simulink subsystem "fft2d"  (R2024b)
settings: Solver=VariableStepAuto  StartTime=0.0  StopTime=10.0  RelTol=1e-3
undefined symbols (not defined in the file): B, L, LOG2B, LOG2L, NFR, PH_W, RAM_AW, W
libraries: hdlsllib x25, dsphdlxfrm2 x1
settings Model: Creator=User  LastModifiedBy=aaala

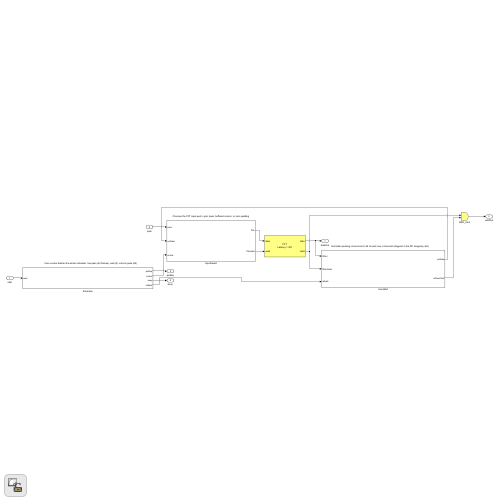
[thumbnail: Simulink's stored preview of the top-level diagram]
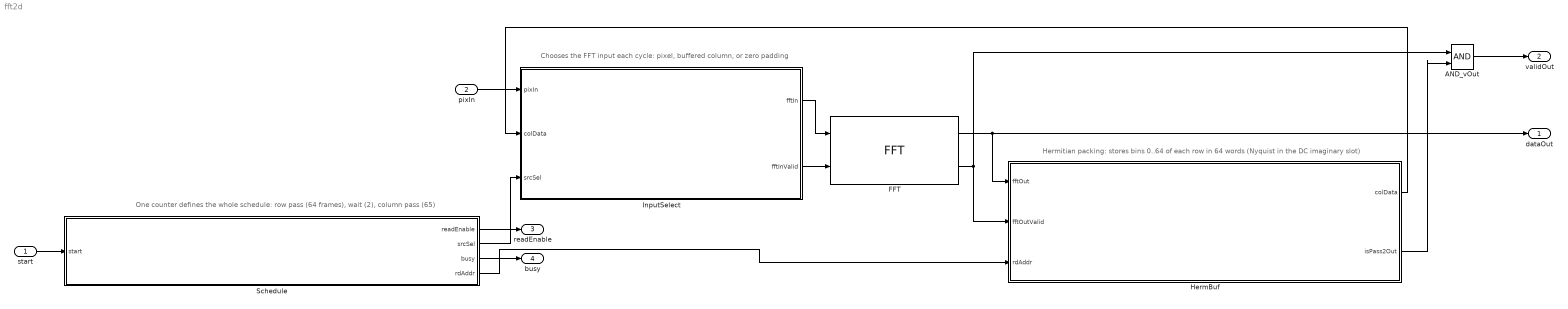
== system fft2d ==
  note: Hermitian packing: stores bins 0..64 of each row in 64 words (Nyquist in the DC imaginary slot)
  note: Chooses the FFT input each cycle: pixel, buffered column, or zero padding
  note: One counter defines the whole schedule: row pass (64 frames), wait (2), column pass (65)
  start : Inport
  pixIn : Inport  Port=2  OutDataTypeStr=uint8
  AND_vOut : Logic  IconShape=distinctive  AllPortsSameDT=off  OutDataTypeStr=boolean
  FFT : dsphdlxfrm2/FFT  Architecture=Streaming Radix 2^2  FFTLengthSource=Property  FFTLength=128  FFTLengthMax=1024  ComplexMultiplication=Use 4 multipliers and 2 adders  BitReversedOutput=off  BitReversedInput=off  Normalize=off  SimulateUsing=Code generation  RoundingMethod=Floor  ResetInputPort=off  StartOutputPort=off  EndOutputPort=off
  HermBuf : Subsystem
  InputSelect : Subsystem
  Schedule : Subsystem
  dataOut : Outport
  validOut : Outport  Port=2
  readEnable : Outport  Port=3
  busy : Outport  Port=4
  wires:
  start/1 -> Schedule/1(start)
  pixIn/1 -> InputSelect/1(pixIn)
  Schedule/3(busy) -> busy/1
  Schedule/1(readEnable) -> readEnable/1
  Schedule/2(srcSel) -> InputSelect/3(srcSel)
  InputSelect/1(fftIn) -> FFT/1
  Schedule/4(rdAddr) -> HermBuf/3(rdAddr)
  InputSelect/2(fftInValid) -> FFT/2
  FFT/1 -> HermBuf/1(fftOut), dataOut/1
  FFT/2 -> HermBuf/2(fftOutValid), AND_vOut/1
  HermBuf/1(colData) -> InputSelect/2(colData)
  HermBuf/2(isPass2Out) -> AND_vOut/2
  AND_vOut/1 -> validOut/1

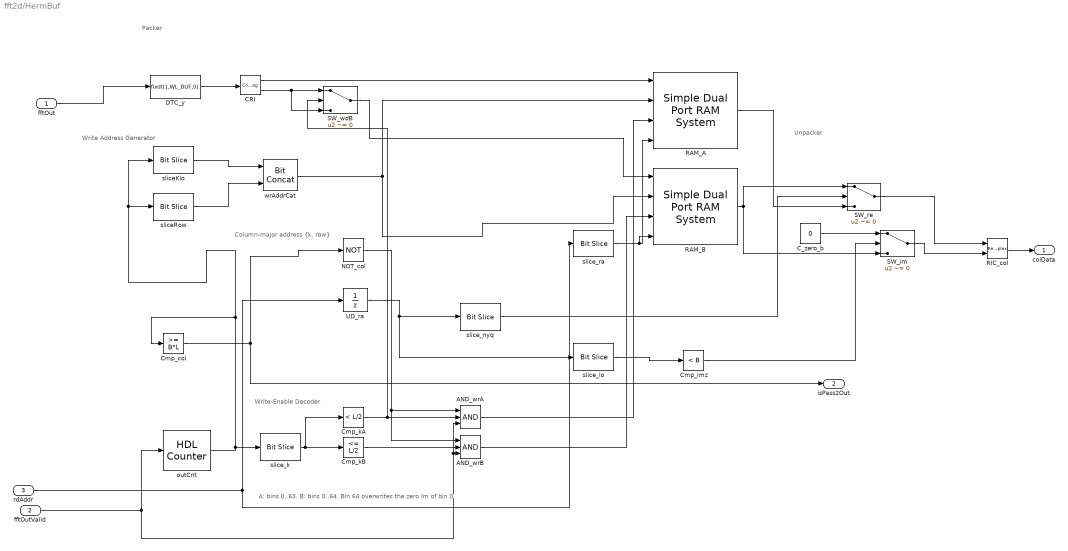
== system fft2d/HermBuf ==
  note: Write-Enable Decoder
  note: A: bins 0..63. B: bins 0..64. Bin 64 overwrites the zero Im of bin 0
  note: Write Address Generator
  note: Column-major address {k, row}
  note: Packer
  note: Unpacker
  fftOut : Inport
  fftOutValid : Inport  Port=2
  rdAddr : Inport  Port=3
  AND_wrA : Logic  Inputs=3  IconShape=distinctive  AllPortsSameDT=off  OutDataTypeStr=boolean
  AND_wrB : Logic  Inputs=3  IconShape=distinctive  AllPortsSameDT=off  OutDataTypeStr=boolean
  CRI : ComplexToRealImag
  C_zero_b : Constant  Value=0  OutDataTypeStr=fixdt(1,WL_BUF,0)
  Cmp_col : hdlsllib/Logic and Bit Operations/Compare To Constant  relop=>=  const=B*L  OutDataTypeStr=boolean
  Cmp_imz : hdlsllib/Logic and Bit Operations/Compare To Constant  relop=<  const=B  OutDataTypeStr=boolean
  Cmp_kA : hdlsllib/Logic and Bit Operations/Compare To Constant  relop=<  const=L/2  OutDataTypeStr=boolean
  Cmp_kB : hdlsllib/Logic and Bit Operations/Compare To Constant  relop=<=  const=L/2  OutDataTypeStr=boolean
  DTC_y : DataTypeConversion  OutDataTypeStr=fixdt(1,WL_BUF,0)  SaturateOnIntegerOverflow=off  RndMeth=Floor
  NOT_col : Logic  Operator=NOT  IconShape=distinctive  AllPortsSameDT=off  OutDataTypeStr=boolean
  RAM_A : hdlsllib/HDL RAMs/Simple Dual Port RAM System  RAMType=Simple dual port  AsyncRead=off  WriteOutputValue=New data  RAMInitialValue=0  allowBusInputs=off  WritesHaveOutput=on  NumReads=0  NumWrites=1  SimulateUsing=Code generation  ModelRAMDelay=on
  RAM_B : hdlsllib/HDL RAMs/Simple Dual Port RAM System  RAMType=Simple dual port  AsyncRead=off  WriteOutputValue=New data  RAMInitialValue=0  allowBusInputs=off  WritesHaveOutput=on  NumReads=0  NumWrites=1  SimulateUsing=Code generation  ModelRAMDelay=on
  RIC_col : RealImagToComplex
  SW_im : Switch  Criteria=u2 ~= 0  SaturateOnIntegerOverflow=off  InputSameDT=off
  SW_re : Switch  Criteria=u2 ~= 0  SaturateOnIntegerOverflow=off  InputSameDT=off
  SW_wdB : Switch  Criteria=u2 ~= 0  SaturateOnIntegerOverflow=off  InputSameDT=off
  UD_ra : UnitDelay  SampleTime=-1  HasFrameUpgradeWarning=on
  outCnt : hdlsllib/Sources/HDL Counter  CountType=Count limited  CountInit=0  CountStep=1  CountMax=OC_MAX  CountFromType=Initial value  CountFrom=0  CountResetPort=off  CountLoadPort=off  CountEnbPort=on  CountDirPort=off  CountHitOutputPort=off  CountDataType=Unsigned  CountWordLen=OC_W  CountFracLen=0  CountSampTime=1
  sliceKlo : hdlsllib/Logic and Bit Operations/Bit Slice  lidx=LOG2L-2  ridx=0
  sliceRow : hdlsllib/Logic and Bit Operations/Bit Slice  lidx=LOG2L+LOG2B-1  ridx=LOG2L
  slice_k : hdlsllib/Logic and Bit Operations/Bit Slice  lidx=LOG2L-1  ridx=0
  slice_lo : hdlsllib/Logic and Bit Operations/Bit Slice  lidx=RAM_AW-1  ridx=0
  slice_nyq : hdlsllib/Logic and Bit Operations/Bit Slice  lidx=RAM_AW  ridx=RAM_AW
  slice_ra : hdlsllib/Logic and Bit Operations/Bit Slice  lidx=RAM_AW-1  ridx=0
  wrAddrCat : hdlsllib/Logic and Bit Operations/Bit Concat  numInputs=2
  colData : Outport
  isPass2Out : Outport  Port=2
  wires:
  SW_im/1 -> RIC_col/2
  SW_re/1 -> RIC_col/1
  Cmp_imz/1 -> SW_im/2
  C_zero_b/1 -> SW_im/1
  RAM_B/1 -> SW_re/1, SW_im/3
  RAM_A/1 -> SW_re/3
  slice_nyq/1 -> SW_re/2
  AND_wrB/1 -> RAM_B/3
  slice_ra/1 -> RAM_B/4, RAM_A/4
  AND_wrA/1 -> RAM_A/3
  RIC_col/1 -> colData/1
  Cmp_kB/1 -> AND_wrB/2
  Cmp_kA/1 -> AND_wrA/2, SW_wdB/2
  wrAddrCat/1 -> RAM_B/2, RAM_A/2
  NOT_col/1 -> AND_wrB/1, AND_wrA/1
  CRI/2 -> SW_wdB/1, SW_wdB/3
  slice_lo/1 -> Cmp_imz/1
  CRI/1 -> RAM_A/1
  UD_ra/1 -> slice_nyq/1, slice_lo/1
  Cmp_col/1 -> isPass2Out/1, NOT_col/1
  slice_k/1 -> Cmp_kA/1, Cmp_kB/1
  DTC_y/1 -> CRI/1
  sliceRow/1 -> wrAddrCat/2
  SW_wdB/1 -> RAM_B/1
  outCnt/1 -> slice_k/1, Cmp_col/1, sliceRow/1, sliceKlo/1
  rdAddr/1 -> UD_ra/1, slice_ra/1
  fftOut/1 -> DTC_y/1
  fftOutValid/1 -> outCnt/1, AND_wrB/3, AND_wrA/3
  sliceKlo/1 -> wrAddrCat/1

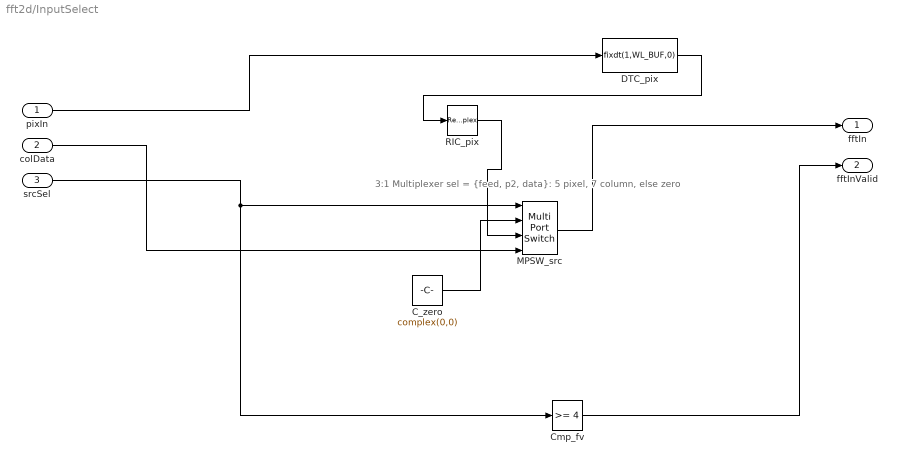
== system fft2d/InputSelect ==
  note: 3:1 Multiplexer
      |
      |
      |
      |
      |
      |
      |
      |
      |
      |
      | sel = {feed, p2, data}: 5 pixel, 7 column, else zero
  pixIn : Inport
  colData : Inport  Port=2
  srcSel : Inport  Port=3
  C_zero : Constant  Value=complex(0,0)  OutDataTypeStr=fixdt(1,WL_BUF,0)
  Cmp_fv : hdlsllib/Logic and Bit Operations/Compare To Constant  relop=>=  const=4  OutDataTypeStr=boolean
  DTC_pix : DataTypeConversion  OutDataTypeStr=fixdt(1,WL_BUF,0)  SaturateOnIntegerOverflow=off  RndMeth=Floor
  MPSW_src : MultiPortSwitch  DataPortOrder=Specify indices  DataPortIndices={[0 1 2 3 4 6], 5, 7}  SaturateOnIntegerOverflow=off  InputSameDT=off
  RIC_pix : RealImagToComplex  Input=Real
  fftIn : Outport
  fftInValid : Outport  Port=2
  wires:
  Cmp_fv/1 -> fftInValid/1
  colData/1 -> MPSW_src/4
  srcSel/1 -> MPSW_src/1, Cmp_fv/1
  MPSW_src/1 -> fftIn/1
  C_zero/1 -> MPSW_src/2
  RIC_pix/1 -> MPSW_src/3
  DTC_pix/1 -> RIC_pix/1
  pixIn/1 -> DTC_pix/1

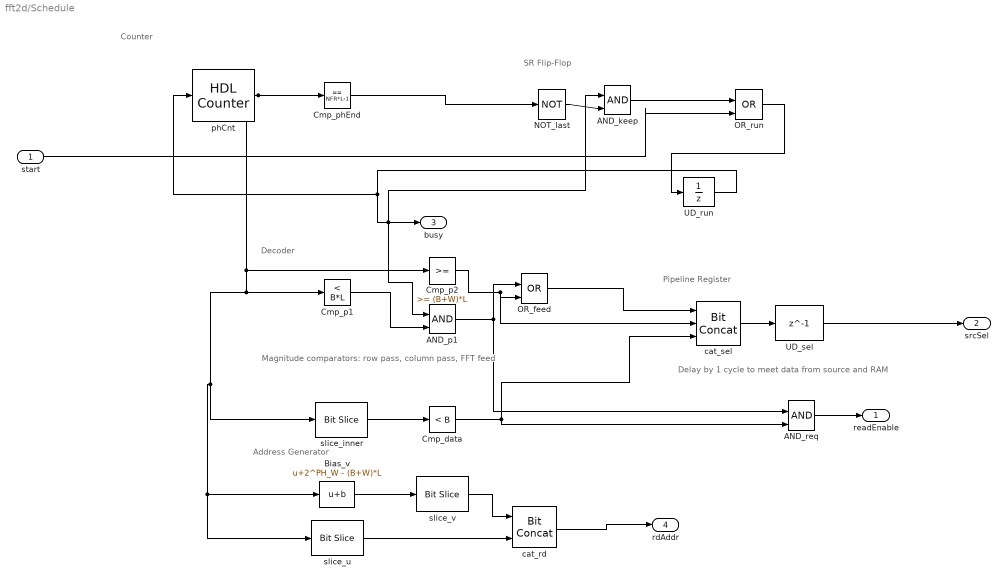
== system fft2d/Schedule ==
  note: SR Flip-Flop
  note: Counter
  note: Decoder
  note: Address Generator
  note: Pipeline Register
  note: Delay by 1 cycle to meet data from source and RAM
  note: Magnitude comparators: row pass, column pass, FFT feed
  start : Inport
  AND_keep : Logic  IconShape=distinctive  AllPortsSameDT=off  OutDataTypeStr=boolean
  AND_p1 : Logic  IconShape=distinctive  AllPortsSameDT=off  OutDataTypeStr=boolean
  AND_req : Logic  IconShape=distinctive  AllPortsSameDT=off  OutDataTypeStr=boolean
  Bias_v : Bias  Bias=2^PH_W - (B+W)*L  SaturateOnIntegerOverflow=off
  Cmp_data : hdlsllib/Logic and Bit Operations/Compare To Constant  relop=<  const=B  OutDataTypeStr=boolean
  Cmp_p1 : hdlsllib/Logic and Bit Operations/Compare To Constant  relop=<  const=B*L  OutDataTypeStr=boolean
  Cmp_p2 : hdlsllib/Logic and Bit Operations/Compare To Constant  relop=>=  const=(B+W)*L  OutDataTypeStr=boolean
  Cmp_phEnd : hdlsllib/Logic and Bit Operations/Compare To Constant  relop===  const=NFR*L-1  OutDataTypeStr=boolean
  NOT_last : Logic  Operator=NOT  IconShape=distinctive  AllPortsSameDT=off  OutDataTypeStr=boolean
  OR_feed : Logic  Operator=OR  IconShape=distinctive  AllPortsSameDT=off  OutDataTypeStr=boolean
  OR_run : Logic  Operator=OR  IconShape=distinctive  AllPortsSameDT=off  OutDataTypeStr=boolean
  UD_run : UnitDelay  SampleTime=-1  HasFrameUpgradeWarning=on
  UD_sel : Delay  DelayLength=1  InitialCondition=0  UseCircularBuffer=on
  cat_rd : hdlsllib/Logic and Bit Operations/Bit Concat  numInputs=2
  cat_sel : hdlsllib/Logic and Bit Operations/Bit Concat  numInputs=3
  phCnt : hdlsllib/Sources/HDL Counter  CountType=Count limited  CountInit=0  CountStep=1  CountMax=NFR*L-1  CountFromType=Initial value  CountFrom=0  CountResetPort=off  CountLoadPort=off  CountEnbPort=on  CountDirPort=off  CountHitOutputPort=off  CountDataType=Unsigned  CountWordLen=PH_W  CountFracLen=0  CountSampTime=1
  slice_inner : hdlsllib/Logic and Bit Operations/Bit Slice  lidx=LOG2L-1  ridx=0
  slice_u : hdlsllib/Logic and Bit Operations/Bit Slice  lidx=LOG2B-1  ridx=0
  slice_v : hdlsllib/Logic and Bit Operations/Bit Slice  lidx=2*LOG2L-1  ridx=LOG2L
  readEnable : Outport
  srcSel : Outport  Port=2
  busy : Outport  Port=3
  rdAddr : Outport  Port=4
  wires:
  UD_sel/1 -> srcSel/1
  cat_sel/1 -> UD_sel/1
  cat_rd/1 -> rdAddr/1
  AND_req/1 -> readEnable/1
  AND_keep/1 -> OR_run/1
  slice_v/1 -> cat_rd/1
  Cmp_data/1 -> AND_req/2, cat_sel/3
  AND_p1/1 -> OR_feed/1, AND_req/1
  Cmp_p2/1 -> OR_feed/2, cat_sel/2
  NOT_last/1 -> AND_keep/2
  Bias_v/1 -> slice_v/1
  slice_u/1 -> cat_rd/2
  start/1 -> OR_run/2
  OR_run/1 -> UD_run/1
  slice_inner/1 -> Cmp_data/1
  OR_feed/1 -> cat_sel/1
  Cmp_p1/1 -> AND_p1/2
  UD_run/1 -> phCnt/1, busy/1, AND_p1/1, AND_keep/1
  Cmp_phEnd/1 -> NOT_last/1
  phCnt/1 -> Cmp_p1/1, Bias_v/1, slice_u/1, slice_inner/1, Cmp_p2/1, Cmp_phEnd/1
